simulink model "BeltStarterGenerator"  (R2024a)
settings: Solver=ode23t  StartTime=0.0  StopTime=0.5  FixedStep=2e-6  RelTol=1e-3  EnableMultiTasking=on
PreLoadFcn:
  | BeltStarterGeneratorData;
undefined symbols (not defined in the file): fswd, Ki_dcdc, Ki_vdc, Kp_dcdc, Kp_vdc, Ld, Lq, p, psim, Tmax, Ts, VDC_VECT
libraries: fl_lib x22, nesl_utility x17, ee_lib x5, eeDiscretePi x3, batteryecm_lib x2, simulink x2, eeTransforms x2, eePmsmCurrentController x1, eePmsmCurrentReferenceGen x1, eePmsmTorqueEstimator x1, eePwmGeneratorTwoLevel x1
(part 1 of 2)
CloseFcn:
  | try,close(h1_BeltStarterGenerator),end
  | clear h1_BeltStarterGenerator
  | 
  | clear simlog_BeltStarterGenerator
  | clear logsout_BeltStarterGenerator
Description:
  | Energy Balance in a 48V Starter Generator
settings Model: Creator=The MathWorks, Inc.  LastModifiedBy=hirah
settings SolverCC: AlgebraicLoopSolver=TrustRegion  MaxZcPerStep=1
settings DataIOCC: MaxDataPoints=110000  ReturnWorkspaceOutputs=off  SignalLoggingName=logsout_BeltStarterGenerator
settings OptimizationCC: ReuseModelBlockBuffer=off  LifeSpan=inf
settings DebuggingCC: UnderspecifiedInitializationDetection=Classic  MergeDetectMultiDrivingBlocksExec=none  MaxConsecutiveZCsMsg=warning  UnconnectedInputMsg=warning  UnconnectedOutputMsg=warning  UnconnectedLineMsg=warning  SFUnexpectedBacktrackingDiag=warning  SFNoUnconditionalDefaultTransitionDiag=warning  SFExecutionAtInitializationDiag=none  ArithmeticOperatorsInVariantConditions=warning
settings ModelReferenceCC: EnableRefExpFcnMdlSchedulingChecks=on
settings SFSimCC: SimUseLocalCustomCode=off  CustomCodeUndefinedFunction=UseInterfaceOnly
settings RTWCC: RTWUseLocalCustomCode=off  GPUComputeCapability=3.5  DLArmComputeVersion=19.05
settings CodeAppCC: StateflowObjectComments=on
settings GRTTargetCC: TargetLangStandard=C89/C90 (ANSI)
settings ConfigComp: CovMetricSettings=dw  CovSaveCumulativeToWorkspaceVar=on  CovSaveSingleToWorkspaceVar=on  CovExternalEMLEnable=off
settings SimscapeCC: SimscapeNormalizeSystem=off  SimscapeLogType=all  SimscapeLogSimulationStatistics=on  SimscapeLogName=simlog_BeltStarterGenerator  SimscapeLogDataHistory=110000

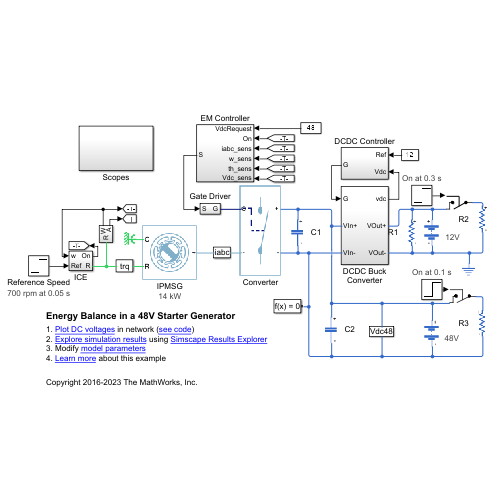
[thumbnail: Simulink's stored preview of the top-level diagram]
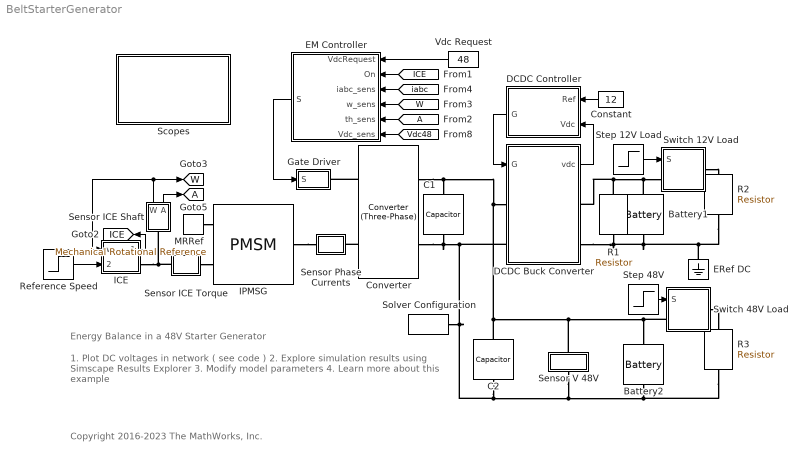
== system BeltStarterGenerator ==
  note: Energy Balance in a 48V Starter Generator
  note: 1. Plot DC voltages in network ( see code )
      | 2. Explore simulation results using Simscape Results Explorer
      | 3. Modify model parameters
      | 4. Learn more about this example
  note: Copyright 2016-2023 The MathWorks, Inc.
  Battery1 : batteryecm_lib/Battery  Vnom=12 V  prm_dir=1  R1_dis=2 Ohm  R1_ch=2 Ohm  R1=0.1 Ohm  prm_AH=1  AH=50 hr*A  V1=11.5 V  AH1=25 hr*A  prm_R2=1  R2=inf Ohm  Tmeas=298.15 K  charge_measurement_port=simscape.enum.battery.enable.no  prm_dyn=1  Rp1=0.005 Ohm  tau1=30 s  Rp2=0.005 Ohm  tau2=30 s  Rp3=0.005 Ohm  tau3=30 s  Rp4=0.005 Ohm  tau4=30 s  Rp5=0.005 Ohm  tau5=30 s  prm_fade=1  N_fade=100  AH_fade=45 hr*A  R1_fade=2.02 Ohm  R1_ch_fade=2.02 Ohm  V1_fade=10.35 V  prm_age=1  prm_age_OCV=1  OCV_age=0.9  SOC_age=60  Tmeas_age=298.15 K  delta_time_age_vec=[0] d  temperature_age_vec=[273] K  OCV_scaling_age=2.2134e6  OCV_offset_age=1.632e6  temp_exp_age=0.515833569 V  t_exp_age=0.75  Vnom_T2=12 V  R1_T2=2.2 Ohm  R1_T2_dis=2.2 Ohm  R1_T2_ch=2.2 Ohm  V1_T2=11.4 V  R2_T2=2200 Ohm  Rp1_T2=0.005 Ohm  tau1_T2=30 s  Rp2_T2=0.005 Ohm  tau2_T2=30 s  Rp3_T2=0.005 Ohm  tau3_T2=30 s  Rp4_T2=0.005 Ohm  tau4_T2=30 s  Rp5_T2=0.005 Ohm  tau5_T2=30 s  Tmeas2=273.15 K  thermal_port=simscape.enum.thermaleffects.omit  thermal_mass=30000 J/K  i_specify=off  i_priority=None  i=0 A  i_nominal_specify=off  i_nominal_value=1  i_nominal_unit=A  v_specify=off  v_priority=None  v=0 V  v_nominal_specify=off  v_nominal_value=1  v_nominal_unit=V  charge_specify=on  charge_priority=High  charge=40 hr*A  charge_nominal_specify=off  charge_nominal_value=1  charge_nominal_unit=A*hr  num_cycles_specify=off  num_cycles_priority=High  num_cycles=0  num_cycles_nominal_specify=off  num_cycles_nominal_value=1  num_cycles_nominal_unit=1  temperature_specify=off  temperature_priority=High  temperature=298.15 K  temperature_nominal_specify=off  temperature_nominal_value=1  temperature_nominal_unit=K
      settings: AttributesFormatString=%<Vnom>%<v_unit>
  Battery2 : batteryecm_lib/Battery  Vnom=48 V  prm_dir=1  R1_dis=2 Ohm  R1_ch=2 Ohm  R1=0.1 Ohm  prm_AH=1  AH=200 hr*A  V1=47 V  AH1=100 hr*A  prm_R2=1  R2=inf Ohm  Tmeas=298.15 K  charge_measurement_port=simscape.enum.battery.enable.no  prm_dyn=1  Rp1=0.005 Ohm  tau1=30 s  Rp2=0.005 Ohm  tau2=30 s  Rp3=0.005 Ohm  tau3=30 s  Rp4=0.005 Ohm  tau4=30 s  Rp5=0.005 Ohm  tau5=30 s  prm_fade=1  N_fade=100  AH_fade=45 hr*A  R1_fade=2.02 Ohm  R1_ch_fade=2.02 Ohm  V1_fade=10.35 V  prm_age=1  prm_age_OCV=1  OCV_age=0.9  SOC_age=60  Tmeas_age=298.15 K  delta_time_age_vec=[0] d  temperature_age_vec=[273] K  OCV_scaling_age=2.2134e6  OCV_offset_age=1.632e6  temp_exp_age=0.515833569 V  t_exp_age=0.75  Vnom_T2=12 V  R1_T2=2.2 Ohm  R1_T2_dis=2.2 Ohm  R1_T2_ch=2.2 Ohm  V1_T2=11.4 V  R2_T2=2200 Ohm  Rp1_T2=0.005 Ohm  tau1_T2=30 s  Rp2_T2=0.005 Ohm  tau2_T2=30 s  Rp3_T2=0.005 Ohm  tau3_T2=30 s  Rp4_T2=0.005 Ohm  tau4_T2=30 s  Rp5_T2=0.005 Ohm  tau5_T2=30 s  Tmeas2=273.15 K  thermal_port=simscape.enum.thermaleffects.omit  thermal_mass=30000 J/K  i_specify=off  i_priority=None  i=0 A  i_nominal_specify=off  i_nominal_value=1  i_nominal_unit=A  v_specify=off  v_priority=None  v=0 V  v_nominal_specify=off  v_nominal_value=1  v_nominal_unit=V  charge_specify=on  charge_priority=High  charge=150 hr*A  charge_nominal_specify=off  charge_nominal_value=1  charge_nominal_unit=A*hr  num_cycles_specify=off  num_cycles_priority=High  num_cycles=0  num_cycles_nominal_specify=off  num_cycles_nominal_value=1  num_cycles_nominal_unit=1  temperature_specify=off  temperature_priority=High  temperature=298.15 K  temperature_nominal_specify=off  temperature_nominal_value=1  temperature_nominal_unit=K
      settings: AttributesFormatString=%<Vnom>%<v_unit>
  C1 : fl_lib/Electrical/Electrical Elements/Capacitor  c=Cdc F  r=1e-6 Ohm  g=0 1/Ohm  i_specify=off  i_priority=None  i=0 A  i_nominal_specify=off  i_nominal_value=1  i_nominal_unit=A  v_specify=on  v_priority=Low  v=50 V  v_nominal_specify=off  v_nominal_value=1  v_nominal_unit=V  vc_specify=on  vc_priority=Low  vc=48 V  vc_nominal_specify=off  vc_nominal_value=1  vc_nominal_unit=V
  C2 : fl_lib/Electrical/Electrical Elements/Capacitor  c=Cdc F  r=1e-6 Ohm  g=0 1/Ohm  i_specify=off  i_priority=None  i=0 A  i_nominal_specify=off  i_nominal_value=1  i_nominal_unit=A  v_specify=on  v_priority=Low  v=50 V  v_nominal_specify=off  v_nominal_value=1  v_nominal_unit=V  vc_specify=on  vc_priority=Low  vc=52 V  vc_nominal_specify=off  vc_nominal_value=1  vc_nominal_unit=V
  Constant : Constant  Value=12  SampleTime=1e-3
  Converter : ee_lib/Semiconductors & Converters/Converters/Converter (Three-Phase)  port_option=ee.enum.threePhasePort.composite  fidelity_option=ee.enum.converters.fidelity.detailed  device_type=2  K=0  Vf=0.8 V  Ron=0.001 Ohm  Rds=0.001 Ohm  Goff=1e-5 1/Ohm  Vgt=1 V  Vgt_off=-1 V  Ih=1 A  Vth=0.5 V  diode_param=2  diode_Vf=0.8 V  diode_Ron=0.001 Ohm  diode_Goff=1e-5 1/Ohm  diode_C=50 nF  diode_iRM=-235 A  diode_iF=300 A  diode_idot=-50 A/us  diode_trr_param=1  diode_trr_factor=3  diode_trr=15 us  diode_Qrr=1.5e+3 s*uA  snubber_type=0  Cs=1e-7 F  Rs=0.1 Ohm
  DCDC Buck Converter : Subsystem  Tag=PublishSubsystem
  DCDC Controller : Subsystem
  EM Controller : Subsystem
  ERef DC : fl_lib/Electrical/Electrical Elements/Electrical Reference
  From2 : From  TagVisibility=global
  Gate Driver : Subsystem
  Goto5 : Goto  TagVisibility=global
  ICE : Subsystem
  IPMSG : ee_lib/Electromechanical/Permanent Magnet/PMSM  port_option=ee.enum.threePhasePort.composite  winding_type=ee.enum.statorconnection.wye  machine_param=ee.enum.pmsm.parameterization.constant  nPolePairs=p  pmflux_param=1  pm_flux_linkage=psim Wb  torque_constant=0.18 N*m/A  back_emf_constant=0.18 V/(rad/s)  stator_param=1  Ld=Ld H  Lq=Lq H  idVec=[-200, 0, 200] A  iqVec=[-200, 0, 200] A  LdMatrix=0.0002 * ones(3, 3) H  LqMatrix=0.0002 * ones(3, 3) H  PmMatrix=0.1 * ones(3, 3) Wb  ktMatrix=0.18 * ones(3, 3) N*m/A  keMatrix=0.18 * ones(3, 3) V/(rad/s)  L0=L0 H  Ls=0.0002 H  Lm=0.00002 H  Ms=0.00002 H  Rs=Rs Ohm  zero_sequence=ee.enum.park.zerosequence.exclude  axes_param=1  loss_param=ee.enum.ironloss.none  losses_oc=[0, 0, 0] W  losses_sc=[0, 0, 0] W  f_losses=60 Hz  Isc_losses=95 A  J=0 kg*m^2  lam=0 N*m/(rad/s)  i_d_specify=off  i_d_priority=None  i_d=0 A  i_d_nominal_specify=off  i_d_nominal_value=1  i_d_nominal_unit=A  i_q_specify=off  i_q_priority=None  i_q=0 A  i_q_nominal_specify=off  i_q_nominal_value=1  i_q_nominal_unit=A  torque_specify=off  torque_priority=None  torque=0 N*m  torque_nominal_specify=off  torque_nominal_value=1  torque_nominal_unit=N*m  angular_velocity_specify=on  angular_velocity_priority=None  angular_velocity=0 rpm  angular_velocity_nominal_specify=off  angular_velocity_nominal_value=1  angular_velocity_nominal_unit=rpm  angular_position_specify=on  angular_position_priority=Low  angular_position=0 rad  angular_position_nominal_specify=off  angular_position_nominal_value=1  angular_position_nominal_unit=deg  alpha=3.93e-3 1/K  alpha_flux=-0.001 1/K  Tmeas=298.15 K  stator_thermal_mass=100 J/K  rotor_thermal_mass=200 J/K  Rm_percent_rotor=90  Rd_percent_rotor=30  temperatureA_specify=off  temperatureA_priority=High  temperatureA=25 degC  temperatureA_nominal_specify=off  temperatureA_nominal_value=1  temperatureA_nominal_unit=degC  temperatureB_specify=off  temperatureB_priority=High  temperatureB=25 degC  temperatureB_nominal_specify=off  temperatureB_nominal_value=1  temperatureB_nominal_unit=degC  temperatureC_specify=off  temperatureC_priority=High  temperatureC=25 degC  temperatureC_nominal_specify=off  temperatureC_nominal_value=1  temperatureC_nominal_unit=degC  temperatureR_specify=off  temperatureR_priority=High  temperatureR=25 degC  temperatureR_nominal_specify=off  temperatureR_nominal_value=1  temperatureR_nominal_unit=degC
      settings: AttributesFormatString=14 kW  InternalSimscapePortConfiguration="{\"Bottom\":[],\"Left\":[{\"id\":\"N\",\"label\":\"~\",\"type\":\"foundation.electrical.three_phase\"}],\"Right\":[{\"id\":\"R\",\"label\":\"R\",\"type\":\"foundation.mechanical.rotational.rotational\"},{\"id\":\"C\",\"label\":\"C\",\"type\":\"foundation.mechanical.rotational.rotational\"}],\"Top\":[]}"
  MRRef : fl_lib/Mechanical/Rotational Elements/Mechanical Rotational Reference
  R1 : fl_lib/Electrical/Electrical Elements/Resistor  R=1 Ohm  i_specify=off  i_priority=None  i=0 A  i_nominal_specify=off  i_nominal_value=1  i_nominal_unit=A  v_specify=off  v_priority=None  v=0 V  v_nominal_specify=off  v_nominal_value=1  v_nominal_unit=V
  R2 : fl_lib/Electrical/Electrical Elements/Resistor  R=1 Ohm  i_specify=off  i_priority=None  i=0 A  i_nominal_specify=off  i_nominal_value=1  i_nominal_unit=A  v_specify=off  v_priority=None  v=0 V  v_nominal_specify=off  v_nominal_value=1  v_nominal_unit=V
  R3 : fl_lib/Electrical/Electrical Elements/Resistor  R=2 Ohm  i_specify=off  i_priority=None  i=0 A  i_nominal_specify=off  i_nominal_value=1  i_nominal_unit=A  v_specify=off  v_priority=None  v=0 V  v_nominal_specify=off  v_nominal_value=1  v_nominal_unit=V
  Reference Speed : Step  Time=0.05  After=700  SampleTime=0
      settings: AttributesFormatString=%<After> rpm at %<Time> s
  Scopes : Subsystem
  Sensor ICE Torque : Subsystem
      mask Display: disp('trq')
  Sensor ICE Shaft : Subsystem
  Sensor Phase Currents : Subsystem
      mask Display: disp('iabc')
  Sensor V 48V : Subsystem
      mask Display: disp('Vdc48')
  Solver Configuration : nesl_utility/Solver Configuration  PhysicalDomain=network_engine_domain  SubClassName=solver  LeftPortType=input  RightPortType=generic  Tones=[]  Harmonics=[]  SimulateNoise=off  Profile=off  UseLocalSampling=off  EnableSwitchedLinearOptims=on  FrequencyDomain=off  UseCCode=off  RelTol=0.001  AbsTol=1e-06  MinStep=1e-09  ToWorkspace=off  RevertToSquareIcSolve=off  NumHomotopyIterations=100  PhasorMode=off  PhasorModeNumHarmonics=1  ConsistencySolver=NEWTON_FTOL  IndexReductionMethod=DerivativeReplacement  DoDC=off  ResidualTolerance=1e-9  ConsistencyTolSource=GLOBAL  ConsistencyAbsTol=0.001  ConsistencyRelTol=0.001  ConsistencyTolFactor=0.001  UseLocalSolver=on  LocalSolverChoice=NE_BACKWARD_EULER_ADVANCER  ResolveIndetEquations=on  FunctionEvalNumThread=1  LocalSolverSampleTime=Ts  DoFixedCost=on  MaxNonlinIter=3  MaxModeIter=2  ComputeImpulses=off  ImpulseIterations=2  LinearAlgebra=auto  LinearAlgebraNumThread=0  EquationFormulation=NE_TIME_EF  DelaysMemoryBudget=1024  AutomaticFiltering=on  FilteringTimeConstant=0.001  PartitionStorageMethod=AS_NEEDED  PartitionMemoryBudget=1024  PartitionMethod=FAST  MultibodyUseLocalSolver=off  MultibodyLocalSolverChoice=ODE1  MultibodyLocalSolverSampleTime=0.001
  Step 12V Load : Step  Time=0.3  SampleTime=0
      settings: AttributesFormatString=On at %<Time> s
  Step 48V : Step  Time=0.1  SampleTime=0
      settings: AttributesFormatString=On at %<Time> s
  Switch 12V Load : Subsystem
      mask Display:
      | patch(-[178.308949107304;178.270428219378;178.155236532808;177.964483406507;177.700005897356;177.364351068347;176.960751458971;176.493093954097;175.965882351142;175.384193986049;174.753630835755;174.080265568098;173.370583058705;172.631417938094;171.869888770445;171.093329497935;170.309218810871;169.525108123807;168.748548851298;167.987019683648;167.247854563037;166.538172053645;165.864806785988;165.234243635694;164.6525552706;164.125343667646;163.657686162771;163.254086553395;162.918431724386;162.653954215236;162.463201088934;162.348009402364;162.309488514438;162.348009402364;162.463201088934;162.653954215236;162.918431724386;163.254086553395;163.657686162771;164.125343667646;164.6525552706;165.234243635694;165.864806785988;166.538172053645;167.247854563037;167.987019683648;168.748548851298;169.525108123807;170.309218810871;171.093329497935;171.869888770445;172.631417938094;173.370583058705;174.080265568098;174.753630835754;175.384193986049;175.965882351142;176.493093954096;176.960751458971;177.364351068347;177.700005897356;177.964483406507;178.155236532808;178.270428219378;178.308949107304;178.308949107304], [113.618216710165;112.834106023101;112.057546750592;111.296017582942;110.556852462331;109.847169952939;109.173804685282;108.543241534988;107.961553169894;107.43434156694;106.966684062065;106.563084452689;106.22742962368;105.962952114529;105.772198988228;105.657007301658;105.618486413732;105.657007301658;105.772198988228;105.962952114529;106.22742962368;106.563084452689;106.966684062065;107.43434156694;107.961553169894;108.543241534988;109.173804685282;109.847169952939;110.556852462331;111.296017582942;112.057546750592;112.834106023101;113.618216710165;114.402327397229;115.178886669738;115.940415837388;116.679580957999;117.389263467392;118.062628735048;118.693191885343;119.274880250436;119.80209185339;120.269749358265;120.673348967641;121.00900379665;121.273481305801;121.464234432102;121.579426118672;121.617947006598;121.579426118672;121.464234432102;121.273481305801;121.00900379665;120.673348967641;120.269749358265;119.80209185339;119.274880250436;118.693191885343;118.062628735048;117.389263467392;116.679580957999;115.940415837388;115.178886669738;114.402327397229;113.618216710165;113.618216710165], [0;0;0])
      | plot(-[178.308949107304;178.270428219378;178.155236532808;177.964483406507;177.700005897356;177.364351068347;176.960751458971;176.493093954097;175.965882351142;175.384193986049;174.753630835755;174.080265568098;173.370583058705;172.631417938094;171.869888770445;171.093329497935;170.309218810871;169.525108123807;168.748548851298;167.987019683648;167.247854563037;166.538172053645;165.864806785988;165.234243635694;164.6525552706;164.125343667646;163.657686162771;163.254086553395;162.918431724386;162.653954215236;162.463201088934;162.348009402364;162.309488514438;162.348009402364;162.463201088934;162.653954215236;162.918431724386;163.254086553395;163.657686162771;164.125343667646;164.6525552706;165.234243635694;165.864806785988;166.538172053645;167.247854563037;167.987019683648;168.748548851298;169.525108123807;170.309218810871;171.093329497935;171.869888770445;172.631417938094;173.370583058705;174.080265568098;174.753630835754;175.384193986049;175.965882351142;176.493093954096;176.960751458971;177.364351068347;177.700005897356;177.964483406507;178.155236532808;178.270428219378;178.308949107304;178.308949107304], [113.618216710165;112.834106023101;112.057546750592;111.296017582942;110.556852462331;109.847169952939;109.173804685282;108.543241534988;107.961553169894;107.43434156694;106.966684062065;106.563084452689;106.22742962368;105.962952114529;105.772198988228;105.657007301658;105.618486413732;105.657007301658;105.772198988228;105.962952114529;106.22742962368;106.563084452689;106.966684062065;107.43434156694;107.961553169894;108.543241534988;109.173804685282;109.847169952939;110.556852462331;111.296017582942;112.057546750592;112.834106023101;113.618216710165;114.402327397229;115.178886669738;115.940415837388;116.679580957999;117.389263467392;118.062628735048;118.693191885343;119.274880250436;119.80209185339;120.269749358265;120.673348967641;121.00900379665;121.273481305801;121.464234432102;121.579426118672;121.617947006598;121.579426118672;121.464234432102;121.273481305801;121.00900379665;120.673348967641;120.269749358265;119.80209185339;119.274880250436;118.693191885343;118.062628735048;117.389263467392;116.679580957999;115.940415837388;115.178886669738;114.402327397229;113.618216710165;113.618216710165])
      | patch(-[64.926944905892;64.888424017966;64.7732323313963;64.5824792050947;64.3180016959439;63.9823468669351;63.5787472575591;63.1110897526843;62.5838781497303;62.0021897846366;61.3716266343423;60.6982613666856;59.988578857293;59.2494137366818;58.4878845690323;57.7113252965232;56.927214609459;56.1431039223949;55.3665446498857;54.6050154822362;53.8658503616251;53.1561678522324;52.4828025845758;51.8522394342815;51.2705510691878;50.7433394662337;50.275681961359;49.872082351983;49.5364275229742;49.2719500138234;49.0811968875218;48.9660052009521;48.9274843130261;48.9660052009521;49.0811968875218;49.2719500138234;49.5364275229742;49.8720823519831;50.275681961359;50.7433394662338;51.2705510691878;51.8522394342816;52.4828025845758;53.1561678522325;53.8658503616251;54.6050154822362;55.3665446498858;56.143103922395;56.927214609459;57.7113252965232;58.4878845690323;59.2494137366818;59.988578857293;60.6982613666856;61.3716266343422;62.0021897846366;62.5838781497303;63.1110897526843;63.5787472575591;63.982346866935;64.3180016959439;64.5824792050947;64.7732323313963;64.888424017966;64.926944905892;64.926944905892], [113.618216710165;112.834106023101;112.057546750592;111.296017582942;110.556852462331;109.847169952939;109.173804685282;108.543241534988;107.961553169894;107.43434156694;106.966684062065;106.563084452689;106.22742962368;105.962952114529;105.772198988228;105.657007301658;105.618486413732;105.657007301658;105.772198988228;105.962952114529;106.22742962368;106.563084452689;106.966684062065;107.43434156694;107.961553169894;108.543241534988;109.173804685282;109.847169952939;110.556852462331;111.296017582942;112.057546750592;112.834106023101;113.618216710165;114.402327397229;115.178886669738;115.940415837388;116.679580957999;117.389263467392;118.062628735048;118.693191885343;119.274880250436;119.80209185339;120.269749358265;120.673348967641;121.00900379665;121.273481305801;121.464234432102;121.579426118672;121.617947006598;121.579426118672;121.464234432102;121.273481305801;121.00900379665;120.673348967641;120.269749358265;119.80209185339;119.274880250436;118.693191885343;118.062628735048;117.389263467392;116.679580957999;115.940415837388;115.178886669738;114.402327397229;113.618216710165;113.618216710165], [0;0;0])
      | plot(-[64.926944905892;64.888424017966;64.7732323313963;64.5824792050947;64.3180016959439;63.9823468669351;63.5787472575591;63.1110897526843;62.5838781497303;62.0021897846366;61.3716266343423;60.6982613666856;59.988578857293;59.2494137366818;58.4878845690323;57.7113252965232;56.927214609459;56.1431039223949;55.3665446498857;54.6050154822362;53.8658503616251;53.1561678522324;52.4828025845758;51.8522394342815;51.2705510691878;50.7433394662337;50.275681961359;49.872082351983;49.5364275229742;49.2719500138234;49.0811968875218;48.9660052009521;48.9274843130261;48.9660052009521;49.0811968875218;49.2719500138234;49.5364275229742;49.8720823519831;50.275681961359;50.7433394662338;51.2705510691878;51.8522394342816;52.4828025845758;53.1561678522325;53.8658503616251;54.6050154822362;55.3665446498858;56.143103922395;56.927214609459;57.7113252965232;58.4878845690323;59.2494137366818;59.988578857293;60.6982613666856;61.3716266343422;62.0021897846366;62.5838781497303;63.1110897526843;63.5787472575591;63.982346866935;64.3180016959439;64.5824792050947;64.7732323313963;64.888424017966;64.926944905892;64.926944905892], [113.618216710165;112.834106023101;112.057546750592;111.296017582942;110.556852462331;109.847169952939;109.173804685282;108.543241534988;107.961553169894;107.43434156694;106.966684062065;106.563084452689;106.22742962368;105.962952114529;105.772198988228;105.657007301658;105.618486413732;105.657007301658;105.772198988228;105.962952114529;106.22742962368;106.563084452689;106.966684062065;107.43434156694;107.961553169894;108.543241534988;109.173804685282;109.847169952939;110.556852462331;111.296017582942;112.057546750592;112.834106023101;113.618216710165;114.402327397229;115.178886669738;115.940415837388;116.679580957999;117.389263467392;118.062628735048;118.693191885343;119.274880250436;119.80209185339;120.269749358265;120.673348967641;121.00900379665;121.273481305801;121.464234432102;121.579426118672;121.617947006598;121.579426118672;121.464234432102;121.273481305801;121.00900379665;120.673348967641;120.269749358265;119.80209185339;119.274880250436;118.693191885343;118.062628735048;117.389263467392;116.679580957999;115.940415837388;115.178886669738;114.402327397229;113.618216710165;113.618216710165])
      | plot(-[56.927214609459;161.805568495765], [113.618216710165;56.927214609459])
      | plot(-[227.000220911577;113.618216710165;113.618216710165], [170.309218810871;170.309218810871;82.4381655547768])
      | patch(-[0;227.23643342033;227.23643342033;0;0;0.472425017505884;0.472425017505884;226.764008402824;226.764008402824;0.472425017505884;0], [227.23643342033;227.23643342033;0;0;227.23643342033;226.764008402824;0.472425017505884;0.472425017505884;226.764008402824;226.764008402824;227.23643342033], [1;1;1])
      | plot(-[170.309218810871;198.654719861224;198.654719861224;227.000220911577], [113.618216710165;113.618216710165;56.927214609459;56.927214609459])
      | plot(-[56.927214609459;0.236212508752942], [113.618216710165;113.618216710165])
  Switch 48V Load : Subsystem
      mask Display:
      | patch(-[178.308949107304;178.270428219378;178.155236532808;177.964483406507;177.700005897356;177.364351068347;176.960751458971;176.493093954097;175.965882351142;175.384193986049;174.753630835755;174.080265568098;173.370583058705;172.631417938094;171.869888770445;171.093329497935;170.309218810871;169.525108123807;168.748548851298;167.987019683648;167.247854563037;166.538172053645;165.864806785988;165.234243635694;164.6525552706;164.125343667646;163.657686162771;163.254086553395;162.918431724386;162.653954215236;162.463201088934;162.348009402364;162.309488514438;162.348009402364;162.463201088934;162.653954215236;162.918431724386;163.254086553395;163.657686162771;164.125343667646;164.6525552706;165.234243635694;165.864806785988;166.538172053645;167.247854563037;167.987019683648;168.748548851298;169.525108123807;170.309218810871;171.093329497935;171.869888770445;172.631417938094;173.370583058705;174.080265568098;174.753630835754;175.384193986049;175.965882351142;176.493093954096;176.960751458971;177.364351068347;177.700005897356;177.964483406507;178.155236532808;178.270428219378;178.308949107304;178.308949107304], [113.618216710165;112.834106023101;112.057546750592;111.296017582942;110.556852462331;109.847169952939;109.173804685282;108.543241534988;107.961553169894;107.43434156694;106.966684062065;106.563084452689;106.22742962368;105.962952114529;105.772198988228;105.657007301658;105.618486413732;105.657007301658;105.772198988228;105.962952114529;106.22742962368;106.563084452689;106.966684062065;107.43434156694;107.961553169894;108.543241534988;109.173804685282;109.847169952939;110.556852462331;111.296017582942;112.057546750592;112.834106023101;113.618216710165;114.402327397229;115.178886669738;115.940415837388;116.679580957999;117.389263467392;118.062628735048;118.693191885343;119.274880250436;119.80209185339;120.269749358265;120.673348967641;121.00900379665;121.273481305801;121.464234432102;121.579426118672;121.617947006598;121.579426118672;121.464234432102;121.273481305801;121.00900379665;120.673348967641;120.269749358265;119.80209185339;119.274880250436;118.693191885343;118.062628735048;117.389263467392;116.679580957999;115.940415837388;115.178886669738;114.402327397229;113.618216710165;113.618216710165], [0;0;0])
      | plot(-[178.308949107304;178.270428219378;178.155236532808;177.964483406507;177.700005897356;177.364351068347;176.960751458971;176.493093954097;175.965882351142;175.384193986049;174.753630835755;174.080265568098;173.370583058705;172.631417938094;171.869888770445;171.093329497935;170.309218810871;169.525108123807;168.748548851298;167.987019683648;167.247854563037;166.538172053645;165.864806785988;165.234243635694;164.6525552706;164.125343667646;163.657686162771;163.254086553395;162.918431724386;162.653954215236;162.463201088934;162.348009402364;162.309488514438;162.348009402364;162.463201088934;162.653954215236;162.918431724386;163.254086553395;163.657686162771;164.125343667646;164.6525552706;165.234243635694;165.864806785988;166.538172053645;167.247854563037;167.987019683648;168.748548851298;169.525108123807;170.309218810871;171.093329497935;171.869888770445;172.631417938094;173.370583058705;174.080265568098;174.753630835754;175.384193986049;175.965882351142;176.493093954096;176.960751458971;177.364351068347;177.700005897356;177.964483406507;178.155236532808;178.270428219378;178.308949107304;178.308949107304], [113.618216710165;112.834106023101;112.057546750592;111.296017582942;110.556852462331;109.847169952939;109.173804685282;108.543241534988;107.961553169894;107.43434156694;106.966684062065;106.563084452689;106.22742962368;105.962952114529;105.772198988228;105.657007301658;105.618486413732;105.657007301658;105.772198988228;105.962952114529;106.22742962368;106.563084452689;106.966684062065;107.43434156694;107.961553169894;108.543241534988;109.173804685282;109.847169952939;110.556852462331;111.296017582942;112.057546750592;112.834106023101;113.618216710165;114.402327397229;115.178886669738;115.940415837388;116.679580957999;117.389263467392;118.062628735048;118.693191885343;119.274880250436;119.80209185339;120.269749358265;120.673348967641;121.00900379665;121.273481305801;121.464234432102;121.579426118672;121.617947006598;121.579426118672;121.464234432102;121.273481305801;121.00900379665;120.673348967641;120.269749358265;119.80209185339;119.274880250436;118.693191885343;118.062628735048;117.389263467392;116.679580957999;115.940415837388;115.178886669738;114.402327397229;113.618216710165;113.618216710165])
      | patch(-[64.926944905892;64.888424017966;64.7732323313963;64.5824792050947;64.3180016959439;63.9823468669351;63.5787472575591;63.1110897526843;62.5838781497303;62.0021897846366;61.3716266343423;60.6982613666856;59.988578857293;59.2494137366818;58.4878845690323;57.7113252965232;56.927214609459;56.1431039223949;55.3665446498857;54.6050154822362;53.8658503616251;53.1561678522324;52.4828025845758;51.8522394342815;51.2705510691878;50.7433394662337;50.275681961359;49.872082351983;49.5364275229742;49.2719500138234;49.0811968875218;48.9660052009521;48.9274843130261;48.9660052009521;49.0811968875218;49.2719500138234;49.5364275229742;49.8720823519831;50.275681961359;50.7433394662338;51.2705510691878;51.8522394342816;52.4828025845758;53.1561678522325;53.8658503616251;54.6050154822362;55.3665446498858;56.143103922395;56.927214609459;57.7113252965232;58.4878845690323;59.2494137366818;59.988578857293;60.6982613666856;61.3716266343422;62.0021897846366;62.5838781497303;63.1110897526843;63.5787472575591;63.982346866935;64.3180016959439;64.5824792050947;64.7732323313963;64.888424017966;64.926944905892;64.926944905892], [113.618216710165;112.834106023101;112.057546750592;111.296017582942;110.556852462331;109.847169952939;109.173804685282;108.543241534988;107.961553169894;107.43434156694;106.966684062065;106.563084452689;106.22742962368;105.962952114529;105.772198988228;105.657007301658;105.618486413732;105.657007301658;105.772198988228;105.962952114529;106.22742962368;106.563084452689;106.966684062065;107.43434156694;107.961553169894;108.543241534988;109.173804685282;109.847169952939;110.556852462331;111.296017582942;112.057546750592;112.834106023101;113.618216710165;114.402327397229;115.178886669738;115.940415837388;116.679580957999;117.389263467392;118.062628735048;118.693191885343;119.274880250436;119.80209185339;120.269749358265;120.673348967641;121.00900379665;121.273481305801;121.464234432102;121.579426118672;121.617947006598;121.579426118672;121.464234432102;121.273481305801;121.00900379665;120.673348967641;120.269749358265;119.80209185339;119.274880250436;118.693191885343;118.062628735048;117.389263467392;116.679580957999;115.940415837388;115.178886669738;114.402327397229;113.618216710165;113.618216710165], [0;0;0])
      | plot(-[64.926944905892;64.888424017966;64.7732323313963;64.5824792050947;64.3180016959439;63.9823468669351;63.5787472575591;63.1110897526843;62.5838781497303;62.0021897846366;61.3716266343423;60.6982613666856;59.988578857293;59.2494137366818;58.4878845690323;57.7113252965232;56.927214609459;56.1431039223949;55.3665446498857;54.6050154822362;53.8658503616251;53.1561678522324;52.4828025845758;51.8522394342815;51.2705510691878;50.7433394662337;50.275681961359;49.872082351983;49.5364275229742;49.2719500138234;49.0811968875218;48.9660052009521;48.9274843130261;48.9660052009521;49.0811968875218;49.2719500138234;49.5364275229742;49.8720823519831;50.275681961359;50.7433394662338;51.2705510691878;51.8522394342816;52.4828025845758;53.1561678522325;53.8658503616251;54.6050154822362;55.3665446498858;56.143103922395;56.927214609459;57.7113252965232;58.4878845690323;59.2494137366818;59.988578857293;60.6982613666856;61.3716266343422;62.0021897846366;62.5838781497303;63.1110897526843;63.5787472575591;63.982346866935;64.3180016959439;64.5824792050947;64.7732323313963;64.888424017966;64.926944905892;64.926944905892], [113.618216710165;112.834106023101;112.057546750592;111.296017582942;110.556852462331;109.847169952939;109.173804685282;108.543241534988;107.961553169894;107.43434156694;106.966684062065;106.563084452689;106.22742962368;105.962952114529;105.772198988228;105.657007301658;105.618486413732;105.657007301658;105.772198988228;105.962952114529;106.22742962368;106.563084452689;106.966684062065;107.43434156694;107.961553169894;108.543241534988;109.173804685282;109.847169952939;110.556852462331;111.296017582942;112.057546750592;112.834106023101;113.618216710165;114.402327397229;115.178886669738;115.940415837388;116.679580957999;117.389263467392;118.062628735048;118.693191885343;119.274880250436;119.80209185339;120.269749358265;120.673348967641;121.00900379665;121.273481305801;121.464234432102;121.579426118672;121.617947006598;121.579426118672;121.464234432102;121.273481305801;121.00900379665;120.673348967641;120.269749358265;119.80209185339;119.274880250436;118.693191885343;118.062628735048;117.389263467392;116.679580957999;115.940415837388;115.178886669738;114.402327397229;113.618216710165;113.618216710165])
      | plot(-[56.927214609459;161.805568495765], [113.618216710165;56.927214609459])
      | plot(-[227.000220911577;113.618216710165;113.618216710165], [170.309218810871;170.309218810871;82.4381655547768])
      | patch(-[0;227.23643342033;227.23643342033;0;0;0.472425017505884;0.472425017505884;226.764008402824;226.764008402824;0.472425017505884;0], [227.23643342033;227.23643342033;0;0;227.23643342033;226.764008402824;0.472425017505884;0.472425017505884;226.764008402824;226.764008402824;227.23643342033], [1;1;1])
      | plot(-[170.309218810871;198.654719861224;198.654719861224;227.000220911577], [113.618216710165;113.618216710165;56.927214609459;56.927214609459])
      | plot(-[56.927214609459;0.236212508752942], [113.618216710165;113.618216710165])
  Vdc Request : Constant  Value=48
  tag scope: ICE=global, W=global
  wires:
  Vdc Request/1 -> EM Controller/1(VdcRequest)
  Step 48V/1 -> Switch 48V Load/1(S)
  DCDC Controller/1(G) -> DCDC Buck Converter/1(G)
  EM Controller/1(S) -> Gate Driver/1(S)
  [Vdc48] -> EM Controller/6(Vdc_sens)
  Sensor ICE Shaft/2(A) -> Goto5/1
  Sensor ICE Shaft/1(W) -> ICE/1(w), [W]
  [W] -> EM Controller/4(w_sens)
  From2/1 -> EM Controller/5(th_sens)
  [iabc] -> EM Controller/3(iabc_sens)
  DCDC Buck Converter/1(vdc) -> DCDC Controller/2(Vdc)
  Reference Speed/1 -> ICE/2(Ref)
  Constant/1 -> DCDC Controller/1(Ref)
  ICE/1(On) -> [ICE]
  [ICE] -> EM Controller/2(On)
  Step 12V Load/1 -> Switch 12V Load/1(S)
  connections:
  Sensor ICE Torque/RConn1 -- ICE/RConn1 -- Sensor ICE Shaft/LConn1
  MRRef/LConn1 -- IPMSG/RConn2
  Converter/LConn1 -- Gate Driver/RConn1
  R1/RConn1 -- ERef DC/LConn1 -- R2/RConn1 -- Battery1/RConn1 -- DCDC Buck Converter/RConn2
  Sensor ICE Torque/LConn1 -- IPMSG/RConn1
  Converter/LConn2 -- Sensor Phase Currents/LConn1
  IPMSG/LConn1 -- Sensor Phase Currents/RConn1
  Switch 48V Load/RConn1 -- R3/LConn1
  Switch 12V Load/RConn1 -- R2/LConn1
  R1/LConn1 -- Battery1/LConn1 -- Switch 12V Load/LConn1 -- DCDC Buck Converter/RConn1
  C2/RConn1 -- R3/RConn1 -- Battery2/RConn1 -- Sensor V 48V/RConn1 -- Solver Configuration/RConn1 -- Converter/RConn2 -- C1/RConn1 -- DCDC Buck Converter/LConn2
  C2/LConn1 -- Converter/RConn1 -- C1/LConn1 -- DCDC Buck Converter/LConn1 -- Sensor V 48V/LConn1 -- Switch 48V Load/LConn1 -- Battery2/LConn1

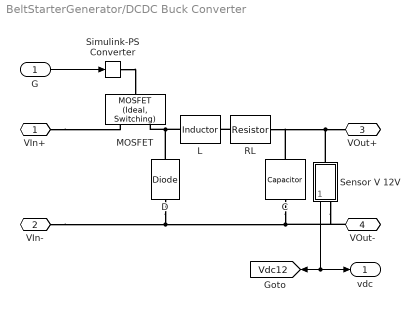
== system BeltStarterGenerator/DCDC Buck Converter ==
  G : Inport
  C : fl_lib/Electrical/Electrical Elements/Capacitor  c=100 uF  r=1e-6 Ohm  g=0 1/Ohm  i_specify=off  i_priority=None  i=0 A  i_nominal_specify=off  i_nominal_value=1  i_nominal_unit=A  v_specify=off  v_priority=None  v=0 V  v_nominal_specify=off  v_nominal_value=1  v_nominal_unit=V  vc_specify=on  vc_priority=Low  vc=0 V  vc_nominal_specify=off  vc_nominal_value=1  vc_nominal_unit=V
  D : fl_lib/Electrical/Electrical Elements/Diode  Vf=0.6 V  Ron=0.3 Ohm  Goff=1e-8 1/Ohm  i_specify=off  i_priority=None  i=0 A  i_nominal_specify=off  i_nominal_value=1  i_nominal_unit=A  v_specify=off  v_priority=None  v=0 V  v_nominal_specify=off  v_nominal_value=1  v_nominal_unit=V
  L : fl_lib/Electrical/Electrical Elements/Inductor  l=3.7 mH  r=0 Ohm  g=1e-9 1/Ohm  i_specify=off  i_priority=None  i=0 A  i_nominal_specify=off  i_nominal_value=1  i_nominal_unit=A  v_specify=off  v_priority=None  v=0 V  v_nominal_specify=off  v_nominal_value=1  v_nominal_unit=V  i_L_specify=on  i_L_priority=Low  i_L=0 A  i_L_nominal_specify=off  i_L_nominal_value=1  i_L_nominal_unit=A
  MOSFET : ee_lib/Semiconductors & Converters/MOSFET (Ideal, Switching)  port_option=ee.enum.controlport.ps  Rds=0.01 Ohm  Goff=1e-6 1/Ohm  Vth=0.5 V  diode_param=2  diode_Vf=0.8 V  diode_Ron=0.001 Ohm  diode_Goff=1e-5 1/Ohm  diode_C=5e-8 F  diode_iRM=-235 A  diode_iF=300 A  diode_idot=-50 A/us  diode_trr_param=1  diode_trr_factor=3  diode_trr=15 us  diode_Qrr=1.5e+3 s*uA  ids_specify=off  ids_priority=None  ids=0 A  ids_nominal_specify=off  ids_nominal_value=1  ids_nominal_unit=A  vds_specify=off  vds_priority=None  vds=0 V  vds_nominal_specify=off  vds_nominal_value=1  vds_nominal_unit=V  vgs_specify=off  vgs_priority=None  vgs=0 V  vgs_nominal_specify=off  vgs_nominal_value=1  vgs_nominal_unit=V  thermal_loss_option=ee.enum.converters.thermalLossOption.constantvalues  Von_data=[0, 1.1, 1.3, 1.45, 1.75, 2.25, 2.7; 0, 1, 1.15, 1.35, 1.7, 2.35, 3] V  Tj=[298.15, 398.15] K  Iout_data=[0, 10, 50, 100, 200, 400, 600] A  Eon_data=[0, .29, 1.43, 2.86, 5.71, 13.14, 22.86; 0, .57, 2.63, 5.14, 10.29, 20.57, 30.29] * 1e-3 J  Eoff_data=[0, .21, 1.07, 2.14, 4.29, 9.86, 17.14; 0, .43, 1.97, 3.86, 7.71, 15.43, 22.71] * 1e-3 J  Eon_data_3D=[zeros(2, 5, 3)] J  Eoff_data_3D=[zeros(2, 5, 3)] J  Tj_loss=[298.15, 398.15] K  Iout_data_loss=[0, 10, 50, 100, 200, 400, 600] A  tabulateWithVds=false  Vds_loss=[0, 150, 300] V  Eon_scalar=22.86e-3 J  Eoff_scalar=17.14e-3 J  Voff=300 V  Iout_scalar=600 A  useCurrentFromPreviousCycle=false  useVoltageFromPreviousCycle=false  diodeModelType=ee.enum.converters.diodeModelType.pwl  diodeTableType=ee.enum.diode.tableType.IfMat  diode_ReverseIVType=ee.enum.diode.diodeReverseIV.constant  diode_IfMat=[.07, .12, .19, 1.75, 4.24, 7.32, 11.2; .16, .3, .72, 2.14, 4.02, 6.35, 9.12] A  diode_VfMat=[.9, 1.15, 1.25, 1.5, 1.75, 2.17, 2.6, 2.85; .58, .68, .75, 1.1, 1.38, 1.77, 2.27, 2.7] V  diode_TjVec=[25, 125] degC  diode_VfVec=[.5, .7, .9, 1.3, 1.7, 2.1, 2.5] V  diode_IfVec=[.1, .2, .5, 1, 2, 4, 7, 10] A  diode_IrMat=[1e-06, 2e-06, 5e-06, 1e-05, 2.5e-05, 5e-05, .0001; 2e-06, 5e-06, 1e-05, 4e-05, 8e-05, .0002, .0005] A  diode_VrMat=[10, 100, 200, 250, 300, 325, 350; 10, 70, 160, 220, 270, 300, 320] V  diode_VrVec=[10, 20, 40, 50, 70, 80, 100] V  diode_IrVec=[1e-06, 2e-06, 5e-06, 1e-05, 2e-05, 5e-05, .0001] A  diode_Vr=-600 V  diode_Ls=150 nH  diode_Erec=0.03 J  diode_rec_loss_model=ee.enum.diode.reverseRecoveryModel.fixed  diode_ErecVal=0 J  diode_scaleWithIandV=true  diode_ErecMat=zeros(2, 3) J  diode_TjrecVec=[298.15, 398.15] K  diode_IfrecVec=[.1, 1, 10] A  diode_IrecVal=10 A  diode_VrecVal=10 V  diode_tFilter=1 / 1000 / 100 s  thermal_network_parameterization=ee.enum.thermalNetworkTopology.external  Rth=[.03, .2] K/W  Rth_Cauer=[.03, .1, .2] K/W  Rth_Foster=[.03, .2] K/W  thermal_mass_parameterization=ee.enum.thermalNetwork.timeconstant  thermal_mass=[3, 25] J/K  thermal_mass_Cauer=[3, 10, 25] J/K  thermal_mass_Foster=[33, 50] J/K  thermal_time_constant=[.1, 5] s  thermal_time_constant_Cauer=[.1, 1, 5] s  thermal_time_constant_Foster=[1, 10] s  thermal_mass_initial_temperatures=[25, 25] degC  thermal_mass_initial_temperatures_Cauer=[25, 25, 25] degC  junction_thermal_mass=0.1 J/K  Tvec_initial_Foster=[25, 25, 25, 25] degC  no_thermal_network=0  junction_temperature_specify=off  junction_temperature_priority=None  junction_temperature=25 degC  junction_temperature_nominal_specify=off  junction_temperature_nominal_value=1  junction_temperature_nominal_unit=degC  Qj_specify=off  Qj_priority=None  Qj=0 W  Qj_nominal_specify=off  Qj_nominal_value=1  Qj_nominal_unit=W  accumulatedSwitchingLosses_specify=off  accumulatedSwitchingLosses_priority=None  accumulatedSwitchingLosses=0 J
  RL : fl_lib/Electrical/Electrical Elements/Resistor  R=1.5 Ohm  i_specify=off  i_priority=None  i=0 A  i_nominal_specify=off  i_nominal_value=1  i_nominal_unit=A  v_specify=off  v_priority=None  v=0 V  v_nominal_specify=off  v_nominal_value=1  v_nominal_unit=V
  Sensor V 12V : Subsystem
  Simulink-PS Converter : nesl_utility/Simulink-PS Converter  PhysicalDomain=network_engine_domain  SubClassName=ps_input  LeftPortType=input  RightPortType=output  PseudoPeriodic=off  Frequencies=[]  NoiseDistribution=none  NoiseParameters=[]  Unit=1  AffineConversion=off  FilteringAndDerivatives=zero  SimscapeFilterOrder=1  InputFilterTimeConstant=0.001  UdotUserProvided=1
  VIn+ : PMIOPort  Side=Left
  VIn- : PMIOPort  Port=2  Side=Left
  VOut+ : PMIOPort  Port=3  Side=Right
  VOut- : PMIOPort  Port=4  Side=Right
  vdc : Outport  VectorParamsAs1DForOutWhenUnconnected=off
  tag scope: Vdc12=global
  wires:
  G/1 -> Simulink-PS Converter/1
  Sensor V 12V/1(vdc) -> [Vdc12], vdc/1
  connections:
  VIn-/RConn1 -- D/LConn1 -- Sensor V 12V/RConn1 -- VOut-/RConn1 -- C/RConn1
  Simulink-PS Converter/RConn1 -- MOSFET/LConn1
  L/LConn1 -- D/RConn1 -- MOSFET/RConn2
  VIn+/RConn1 -- MOSFET/RConn1
  RL/LConn1 -- L/RConn1
  C/LConn1 -- RL/RConn1 -- VOut+/RConn1 -- Sensor V 12V/LConn1

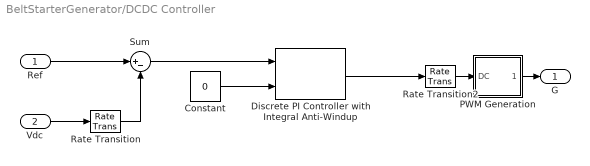
== system BeltStarterGenerator/DCDC Controller ==
  Ref : Inport
  Vdc : Inport  Port=2
  Constant : Constant  Value=0  SampleTime=-1
  Discrete PI Controller with Integral Anti-Windup : eeDiscretePi/Discrete PI Controller with Integral Anti-Windup  Kp=Kp_dcdc  Ki=Ki_dcdc  x0=0  B=1  A=0  Ts=1e-3
  PWM Generation : Subsystem  mask{f=fswd, Ts=Ts}
      mask prompts: f "Switching frequency"; Ts "Sample time"
  Rate Transition : RateTransition  OutPortSampleTime=1e-3
  Rate Transition2 : RateTransition
  Sum : Sum  Inputs=|+-
  G : Outport  VectorParamsAs1DForOutWhenUnconnected=off
  wires:
  Vdc/1 -> Rate Transition/1
  Rate Transition2/1 -> PWM Generation/1(DC)
  Ref/1 -> Sum/1
  Rate Transition/1 -> Sum/2
  PWM Generation/1(PWM) -> G/1
  Sum/1 -> Discrete PI Controller with Integral Anti-Windup/1
  Discrete PI Controller with Integral Anti-Windup/1 -> Rate Transition2/1
  Constant/1 -> Discrete PI Controller with Integral Anti-Windup/2

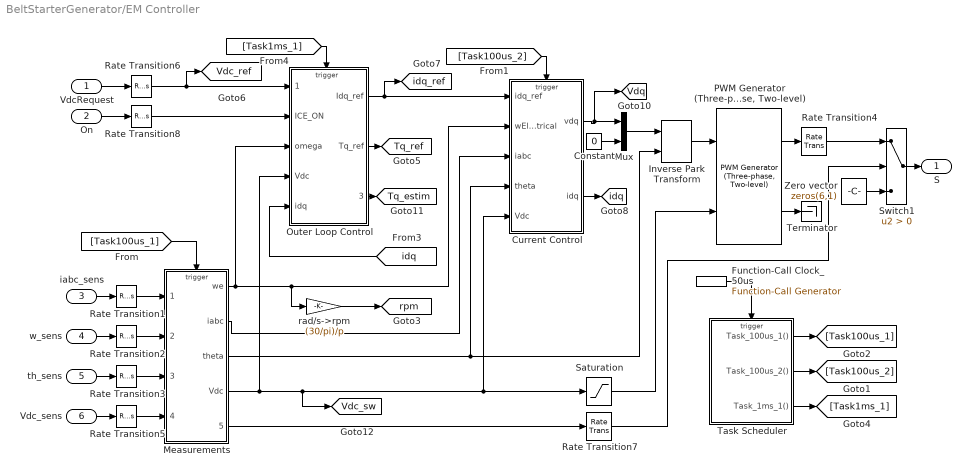
== system BeltStarterGenerator/EM Controller ==
  VdcRequest : Inport
  On : Inport  Port=2
  iabc_sens : Inport  Port=3
  w_sens : Inport  Port=4
  th_sens : Inport  Port=5
  Vdc_sens : Inport  Port=6
  Constant : Constant  Value=0  SampleTime=-1
  Current Control : Subsystem
  Function-Call Clock_50us : simulink/Ports & Subsystems/Function-Call Generator  sample_time=5e-5  numberOfIterations=1  DisallowWideOutput=off
  Inverse Park Transform : eeTransforms/Inverse Park Transform  AxisAlignment=Q-axis  PowerInvariant=off
  Measurements : Subsystem
  Mux : Mux  Inputs=2
  Outer Loop Control : Subsystem
  "PWM Generator (Three-phase, Two-level)" : eePwmGeneratorTwoLevel/PWM Generator (Three-phase, Two-level)  PWMMode=Continuous PWM (CPWM)  CPWMMode=SVM: space vector modulation  DPWMMode=60 DPWM: 60 degree discontinuous PWM  fsw=fsw  Ts=Ts
  Rate Transition{1..8} (8 alike) : RateTransition
  Saturation : Saturate  UpperLimit=500  LowerLimit=10
  Switch1 : Switch  Criteria=u2 > Threshold  SaturateOnIntegerOverflow=off  InputSameDT=off
  Task Scheduler : Stateflow chart  TreatAsAtomicUnit=on
  Terminator : Terminator
  Zero vector : Constant  Value=zeros(6,1)
  rad/s->rpm : Gain  Gain=(30/pi)/p
  S : Outport  VectorParamsAs1DForOutWhenUnconnected=off
  tag scope: Tq_estim=global, Tq_ref=global, Vdc_ref=global, Vdc_sw=global, Vdq=global, idq=global, idq_ref=global, rpm=global
  wires:
  Measurements/4(Vdc) -> Outer Loop Control/4(Vdc), [Vdc_sw], Current Control/5(Vdc), Saturation/1
  [Task1ms_1] -> Outer Loop Control/Trigger
  Rate Transition8/1 -> Outer Loop Control/2(ICE_ON)
  Rate Transition1/1 -> Measurements/1(iabc_sens)
  Switch1/1 -> S/1
  Rate Transition5/1 -> Measurements/4(Vdc_sens)
  Current Control/1(vdq) -> [Vdq], Mux/1
  [idq] -> Outer Loop Control/5(idq)
  Outer Loop Control/1(Idq_ref) -> Current Control/1(idq_ref), [idq_ref]
  Task Scheduler/1(Task_100us_1()) -> [Task100us_1]
  Measurements/3(theta) -> Current Control/4(theta), Inverse Park Transform/2
  Rate Transition4/1 -> Switch1/1
  Outer Loop Control/3(Tq_estim) -> [Tq_estim]
  Rate Transition7/1 -> Switch1/2
  VdcRequest/1 -> Rate Transition6/1
  Zero vector/1 -> Switch1/3
  Measurements/1(we) -> Outer Loop Control/3(omega), rad/s->rpm/1, Current Control/2(wElectrical)
  th_sens/1 -> Rate Transition3/1
  Current Control/2(idq) -> [idq]
  On/1 -> Rate Transition8/1
  Outer Loop Control/2(Tq_ref) -> [Tq_ref]
  Rate Transition6/1 -> Outer Loop Control/1(Vdc_ref), [Vdc_ref]
  iabc_sens/1 -> Rate Transition1/1
  Task Scheduler/3(Task_1ms_1()) -> [Task1ms_1]
  Rate Transition3/1 -> Measurements/3(th_sens)
  Function-Call Clock_50us/1 -> Task Scheduler/Trigger
  Measurements/5(PwmEnable) -> Rate Transition7/1
  "PWM Generator (Three-phase, Two-level)"/2 -> Terminator/1
  Rate Transition2/1 -> Measurements/2(w_sens)
  Saturation/1 -> "PWM Generator (Three-phase, Two-level)"/2
  [Task100us_2] -> Current Control/Trigger
  w_sens/1 -> Rate Transition2/1
  rad/s->rpm/1 -> [rpm]
  Inverse Park Transform/1 -> "PWM Generator (Three-phase, Two-level)"/1
  "PWM Generator (Three-phase, Two-level)"/1 -> Rate Transition4/1
  Vdc_sens/1 -> Rate Transition5/1
  Task Scheduler/2(Task_100us_2()) -> [Task100us_2]
  [Task100us_1] -> Measurements/Trigger
  Measurements/2(iabc) -> Current Control/3(iabc)
  Mux/1 -> Inverse Park Transform/1
  Constant/1 -> Mux/2

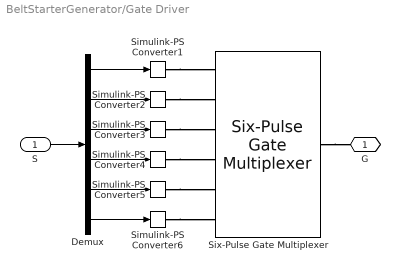
== system BeltStarterGenerator/Gate Driver ==
  S : Inport
  Demux : Demux  Outputs=6
  Simulink-PS Converter{1..6} (6 alike) : nesl_utility/Simulink-PS Converter  PhysicalDomain=network_engine_domain  SubClassName=ps_input  LeftPortType=input  RightPortType=output  PseudoPeriodic=off  Frequencies=[]  NoiseDistribution=none  NoiseParameters=[]  Unit=1  AffineConversion=off  FilteringAndDerivatives=zero  SimscapeFilterOrder=1  InputFilterTimeConstant=0.001  UdotUserProvided=1
  Six-Pulse Gate Multiplexer : ee_lib/Semiconductors & Converters/Converters/Six-Pulse Gate Multiplexer  port_option=ee.enum.controlport.ps
  G : PMIOPort  Side=Right
  wires:
  Demux/1 -> Simulink-PS Converter1/1
  S/1 -> Demux/1
  Demux/4 -> Simulink-PS Converter4/1
  Demux/2 -> Simulink-PS Converter2/1
  Demux/3 -> Simulink-PS Converter3/1
  Demux/5 -> Simulink-PS Converter5/1
  Demux/6 -> Simulink-PS Converter6/1
  connections:
  Six-Pulse Gate Multiplexer/RConn1 -- G/RConn1
  Simulink-PS Converter1/RConn1 -- Six-Pulse Gate Multiplexer/LConn1
  Simulink-PS Converter3/RConn1 -- Six-Pulse Gate Multiplexer/LConn3
  Simulink-PS Converter5/RConn1 -- Six-Pulse Gate Multiplexer/LConn5
  Simulink-PS Converter6/RConn1 -- Six-Pulse Gate Multiplexer/LConn6
  Simulink-PS Converter4/RConn1 -- Six-Pulse Gate Multiplexer/LConn4
  Simulink-PS Converter2/RConn1 -- Six-Pulse Gate Multiplexer/LConn2

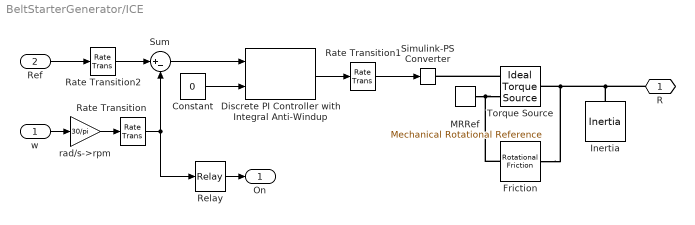
== system BeltStarterGenerator/ICE ==
  w : Inport
  Ref : Inport  Port=2
  Constant : Constant  Value=0  SampleTime=0.01
  Discrete PI Controller with Integral Anti-Windup : eeDiscretePi/Discrete PI Controller with Integral Anti-Windup  Kp=1  Ki=0.8  x0=0  B=50  A=-50  Ts=0.001
  Friction : fl_lib/Mechanical/Rotational Elements/Rotational Friction  brkwy_trq=0.02e-3 N*m  brkwy_vel=0.1 rad/s  Col_trq=0.02e-3 N*m  visc_coef=0.001 N*m/(rad/s)  w_specify=off  w_priority=None  w=0 rad/s  w_nominal_specify=off  w_nominal_value=1  w_nominal_unit=rad/s  t_specify=off  t_priority=None  t=0 N*m  t_nominal_specify=off  t_nominal_value=1  t_nominal_unit=N*m
  Inertia : fl_lib/Mechanical/Rotational Elements/Inertia  inertia=0.02 kg*m^2  num_ports=foundation.enum.numPorts2.one  w_specify=on  w_priority=Low  w=0 rad/s  w_nominal_specify=off  w_nominal_value=1  w_nominal_unit=rad/s  t_specify=off  t_priority=None  t=0 N*m  t_nominal_specify=off  t_nominal_value=1  t_nominal_unit=N*m
  MRRef : fl_lib/Mechanical/Rotational Elements/Mechanical Rotational Reference
  Rate Transition : RateTransition  OutPortSampleTime=0.001
  Rate Transition1 : RateTransition
  Rate Transition2 : RateTransition  OutPortSampleTime=0.001
  Relay : Relay  OnSwitchValue=700  OffSwitchValue=500
  Simulink-PS Converter : nesl_utility/Simulink-PS Converter  PhysicalDomain=network_engine_domain  SubClassName=ps_input  LeftPortType=input  RightPortType=output  PseudoPeriodic=off  Frequencies=[]  NoiseDistribution=none  NoiseParameters=[]  Unit=N*m  AffineConversion=off  FilteringAndDerivatives=zero  SimscapeFilterOrder=1  InputFilterTimeConstant=0.001  UdotUserProvided=1
  Sum : Sum  Inputs=|+-
  Torque Source : fl_lib/Mechanical/Mechanical Sources/Ideal Torque Source
  rad/s->rpm : Gain  Gain=30/pi
  R : PMIOPort  Side=Right
  On : Outport  VectorParamsAs1DForOutWhenUnconnected=off
  wires:
  Rate Transition1/1 -> Simulink-PS Converter/1
  rad/s->rpm/1 -> Rate Transition/1
  Relay/1 -> On/1
  w/1 -> rad/s->rpm/1
  Ref/1 -> Rate Transition2/1
  Rate Transition/1 -> Relay/1, Sum/2
  Sum/1 -> Discrete PI Controller with Integral Anti-Windup/1
  Discrete PI Controller with Integral Anti-Windup/1 -> Rate Transition1/1
  Constant/1 -> Discrete PI Controller with Integral Anti-Windup/2
  Rate Transition2/1 -> Sum/1
  connections:
  R/RConn1 -- Inertia/LConn1 -- Torque Source/LConn1 -- Friction/LConn1
  MRRef/LConn1 -- Friction/RConn1 -- Torque Source/RConn2
  Torque Source/RConn1 -- Simulink-PS Converter/RConn1
